simulink model "Ejercicio_2_3"  (R2026b)
settings: Solver=VariableStepAuto  StopTime=40.0
InitFcn:
  | caso_run = '2.3'; pv_params; clear caso_run
values from neighbouring files (symbols this model uses):
  alpha0 = fzero(f, [0 1])    [pv_params(1).m]    (also in pv_params(2).m; pv_params(3).m; pv_params(4).m; pv_params.m)
  comedelay = 20e-3    (= 0.02)    [pv_params(1).m]    (also in pv_params(2).m; pv_params(3).m; pv_params(4).m; pv_params.m)
  Pavail = [500 500 2000 2000 2000]    [pv_params(1).m]    (also in pv_params(2).m; pv_params(3).m; pv_params(4).m; pv_params.m)
  Pinv_nom = 2000    [pv_params(1).m]    (also in pv_params(2).m; pv_params(3).m; pv_params(4).m; pv_params.m)
  Ppcc0 = sum(min(alpha0*Pinv_nom, Pavail))    [pv_params(1).m]    (also in pv_params(2).m; pv_params(3).m; pv_params(4).m; pv_params.m)
  t_sample_ppc = 0.2    [pv_params(1).m]    (also in pv_params(2).m; pv_params(3).m; pv_params(4).m; pv_params.m)
  t_step = 10    [pv_params(1).m]    (also in pv_params(2).m; pv_params(3).m; pv_params(4).m; pv_params.m)
  tau_pv = 0.5    [pv_params(1).m]    (also in pv_params(2).m; pv_params(3).m; pv_params(4).m; pv_params.m)
settings Model: Creator=mithu  LastModifiedBy=ArnauCoronado

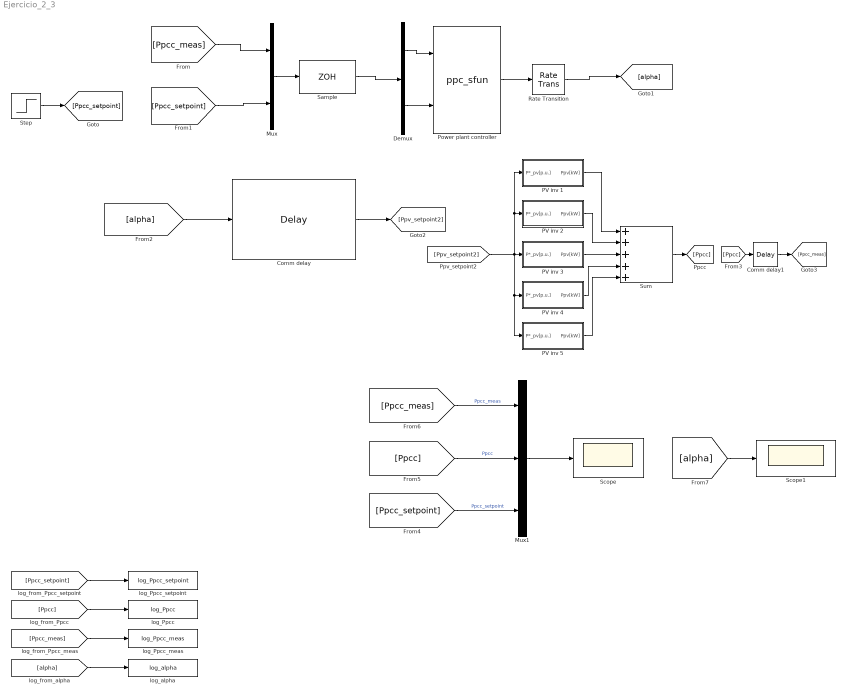
== system Ejercicio_2_3 ==
  Comm delay : TransportDelay  DelayTime=comedelay  InitialOutput=alpha0
  Comm delay1 : TransportDelay  DelayTime=comedelay  InitialOutput=Ppcc0
  Demux : Demux  Outputs=2
  Mux : Mux  Inputs=2
  Mux1 : Mux  Inputs=3
  PV inv 1 : Subsystem
  PV inv 2 : Subsystem
  PV inv 3 : Subsystem
  PV inv 4 : Subsystem
  PV inv 5 : Subsystem
  Power plant controller : M-S-Function  FunctionName=ppc_sfun  Parameters=t_sample_ppc, Kp, Ki, Ppv_nom, ppc_mode, I0
  Rate Transition : RateTransition  Integrity=off  InitialCondition=alpha0
  Sample : ZeroOrderHold  SampleTime=t_sample_ppc
  Scope : Scope
      settings: ActiveDisplayYMinimum=4584.0979177394447  ActiveDisplayYMaximum=7622.8635427394447
  Scope1 : Scope
      settings: ActiveDisplayYMinimum=0.49358086124458955  ActiveDisplayYMaximum=0.72293545986171237
  Step : Step  Time=t_step  InitialValue=P_tso_0  FinalValue=P_tso_1  SampleTime=0
  Sum : Sum  Inputs=+++++
  log_Ppcc : ToWorkspace  VariableName=log_Ppcc  SaveFormat=Timeseries  SampleTime=-1
  log_Ppcc_meas : ToWorkspace  VariableName=log_Ppcc_meas  SaveFormat=Timeseries  SampleTime=-1
  log_Ppcc_setpoint : ToWorkspace  VariableName=log_Ppcc_setpoint  SaveFormat=Timeseries  SampleTime=-1
  log_alpha : ToWorkspace  VariableName=log_alpha  SaveFormat=Timeseries  SampleTime=-1
  wires:
  Step/1 -> [Ppcc_setpoint]
  [Ppcc_meas] -> Mux/1
  [Ppcc_setpoint] -> Mux/2
  Mux/1 -> Sample/1
  Sample/1 -> Demux/1
  Demux/1 -> Power plant controller/1
  Demux/2 -> Power plant controller/2
  Power plant controller/1 -> Rate Transition/1
  Rate Transition/1 -> [alpha]
  [alpha] -> Comm delay/1
  Comm delay/1 -> [Ppv_setpoint2]
  [Ppv_setpoint2] -> PV inv 1/1(P*_pv[p.u.]), PV inv 2/1(P*_pv[p.u.]), PV inv 5/1(P*_pv[p.u.]), PV inv 4/1(P*_pv[p.u.]), PV inv 3/1(P*_pv[p.u.])
  PV inv 1/1(Ppv[kW]) -> Sum/1
  PV inv 3/1(Ppv[kW]) -> Sum/3
  PV inv 4/1(Ppv[kW]) -> Sum/4
  PV inv 5/1(Ppv[kW]) -> Sum/5
  PV inv 2/1(Ppv[kW]) -> Sum/2
  Sum/1 -> [Ppcc]
  [Ppcc] -> Comm delay1/1
  Comm delay1/1 -> [Ppcc_meas]
  [Ppcc_meas] -> Mux1/1  "Ppcc_meas"
  [Ppcc] -> Mux1/2  "Ppcc"
  [Ppcc_setpoint] -> Mux1/3  "Ppcc_setpoint"
  Mux1/1 -> Scope/1
  [alpha] -> Scope1/1
  [Ppcc_setpoint] -> log_Ppcc_setpoint/1
  [Ppcc] -> log_Ppcc/1
  [Ppcc_meas] -> log_Ppcc_meas/1
  [alpha] -> log_alpha/1

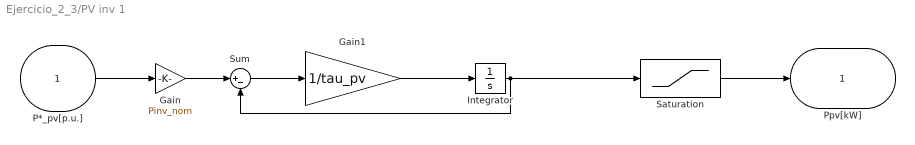
== system Ejercicio_2_3/PV inv 1 ==
  P*_pv[p.u.] : Inport
  Gain : Gain  Gain=Pinv_nom
  Gain1 : Gain  Gain=1/tau_pv
  Integrator : Integrator  InitialCondition=alpha0*Pinv_nom
  Saturation : Saturate  UpperLimit=Pavail(1)  LowerLimit=0
  Sum : Sum  Inputs=|+-
  Ppv[kW] : Outport
  wires:
  Saturation/1 -> Ppv[kW]/1
  P*_pv[p.u.]/1 -> Gain/1
  Gain/1 -> Sum/1
  Sum/1 -> Gain1/1
  Gain1/1 -> Integrator/1
  Integrator/1 -> Saturation/1, Sum/2

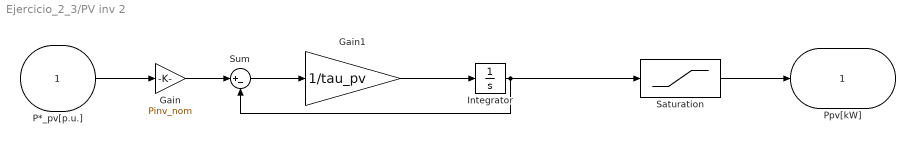
== system Ejercicio_2_3/PV inv 2 ==
  P*_pv[p.u.] : Inport
  Gain : Gain  Gain=Pinv_nom
  Gain1 : Gain  Gain=1/tau_pv
  Integrator : Integrator  InitialCondition=alpha0*Pinv_nom
  Saturation : Saturate  UpperLimit=Pavail(2)  LowerLimit=0
  Sum : Sum  Inputs=|+-
  Ppv[kW] : Outport
  wires:
  P*_pv[p.u.]/1 -> Gain/1
  Gain/1 -> Sum/1
  Sum/1 -> Gain1/1
  Gain1/1 -> Integrator/1
  Integrator/1 -> Saturation/1, Sum/2
  Saturation/1 -> Ppv[kW]/1

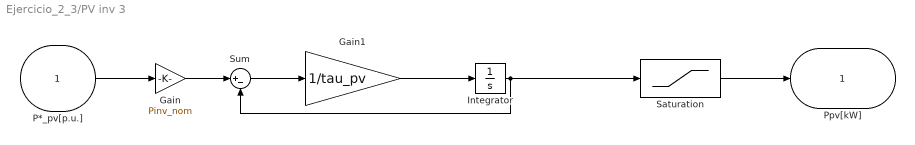
== system Ejercicio_2_3/PV inv 3 ==
  P*_pv[p.u.] : Inport
  Gain : Gain  Gain=Pinv_nom
  Gain1 : Gain  Gain=1/tau_pv
  Integrator : Integrator  InitialCondition=alpha0*Pinv_nom
  Saturation : Saturate  UpperLimit=Pavail(3)  LowerLimit=0
  Sum : Sum  Inputs=|+-
  Ppv[kW] : Outport
  wires:
  P*_pv[p.u.]/1 -> Gain/1
  Gain/1 -> Sum/1
  Sum/1 -> Gain1/1
  Gain1/1 -> Integrator/1
  Integrator/1 -> Saturation/1, Sum/2
  Saturation/1 -> Ppv[kW]/1

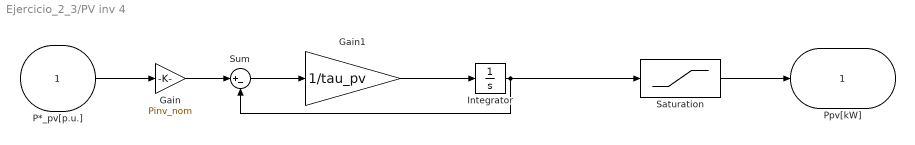
== system Ejercicio_2_3/PV inv 4 ==
  P*_pv[p.u.] : Inport
  Gain : Gain  Gain=Pinv_nom
  Gain1 : Gain  Gain=1/tau_pv
  Integrator : Integrator  InitialCondition=alpha0*Pinv_nom
  Saturation : Saturate  UpperLimit=Pavail(4)  LowerLimit=0
  Sum : Sum  Inputs=|+-
  Ppv[kW] : Outport
  wires:
  P*_pv[p.u.]/1 -> Gain/1
  Gain/1 -> Sum/1
  Sum/1 -> Gain1/1
  Gain1/1 -> Integrator/1
  Integrator/1 -> Saturation/1, Sum/2
  Saturation/1 -> Ppv[kW]/1

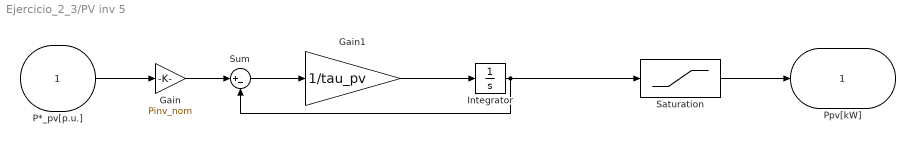
== system Ejercicio_2_3/PV inv 5 ==
  P*_pv[p.u.] : Inport
  Gain : Gain  Gain=Pinv_nom
  Gain1 : Gain  Gain=1/tau_pv
  Integrator : Integrator  InitialCondition=alpha0*Pinv_nom
  Saturation : Saturate  UpperLimit=Pavail(5)  LowerLimit=0
  Sum : Sum  Inputs=|+-
  Ppv[kW] : Outport
  wires:
  P*_pv[p.u.]/1 -> Gain/1
  Gain/1 -> Sum/1
  Sum/1 -> Gain1/1
  Gain1/1 -> Integrator/1
  Integrator/1 -> Saturation/1, Sum/2
  Saturation/1 -> Ppv[kW]/1
